simulink model "r2_b16a4x64f"  (R2012b)
settings: Solver=VariableStepDiscrete  SolverMode=SingleTasking  StartTime=0.0  StopTime=1  RelTol=1e-3
undefined symbols (not defined in the file): fft_stages, n_bits_ants, n_bits_xengs
libraries: xbsIndex_r4 x26846, casper_library_misc x230, xbsReplacements_r4 x24, casper_library_delays x8, xps_library x5, casper_library_communications x4
(part 37 of 227)

== system r2_b16a4x64f/sys0/xeng ==
  sync_in : Inport
  ant : Inport  Port=2
  window_valid : Inport  Port=3
  mcnt_in : Inport  Port=4
  Constant : xbsIndex_r4/Constant  const=0  gui_display_data_type=Fixed-point  arith_type=Unsigned  n_bits=200  bin_pt=14  preci_type=Single  exp_width=8  frac_width=24  explicit_period=on  period=1  equ=P=C  opselect=C  inp2=PCIN>>17  opr=+  inp1=P  carry=CIN  dbl_ovrd=off  block_type=constant
  Constant1 : xbsIndex_r4/Constant  const=0  gui_display_data_type=Fixed-point  arith_type=Boolean  n_bits=1  bin_pt=14  preci_type=Single  exp_width=8  frac_width=24  explicit_period=on  period=1  equ=P=C  opselect=C  inp2=PCIN>>17  opr=+  inp1=P  carry=CIN  dbl_ovrd=off  block_type=constant
  Term1 : Terminator
  Term2 : Terminator
  Term3 : Terminator
  auto_tap : Subsystem  AncestorBlock=casper_library_correlator/auto_tap  mask(auto_tap){n_ants=16, n_simultan=2, n_bits=8, acc_len=256, add_latency=3, mult_latency=4, bram_latency=7, mult_type=1, use_bram_delay=1}
      mask prompts: n_ants "Number of antennas (total inputs = n_ants*n_simultan below)"; n_simultan "Number of inputs fed-in simultaneously"; n_bits "Number of input bits (per complex component)"; acc_len "Accumulation length"; add_latency "Adder latency"; mult_latency "Multiplier latency"; bram_latency "BRAM latency"; mult_type "Multiplier Type (0=behavioural HDL, 1=embedded, 2=core)"; use_bram_delay "Implementation: Delay type (0=SLR, 1=BRAM)"
      mask init:
      | fix_pnt_pos = (n_bits-1)*2;
      | bit_growth = ceil(log2(acc_len));
      | ant_bits = ceil(log2(n_ants));
      | n_bits_out = (2*n_bits + 1 + bit_growth);
      | 
      | params = get_mask_params(gcb);
      | auto_tap_init(gcb, params{:});
      settings: AttributesFormatString=mult_typ=1, del_typ=1
  baseline_tap1 : Subsystem  AncestorBlock=casper_library_correlator/baseline_tap  mask(baseline_tap){n_ants=16, ant_sep=1, n_bits=8, acc_len=256, add_latency=3, mult_latency=4, bram_latency=7, mult_type=1, use_bram_delay=1}
      mask prompts: n_ants "Number of antennas"; ant_sep "Antenna Seperation"; n_bits "number of input bits (per complex component)"; acc_len "accumulation length"; add_latency "Adder latency"; mult_latency "Multiplier latency"; bram_latency "BRAM latency"; mult_type "Multiplier Type (0=behavioural HDL, 1=embedded, 2=core)"; use_bram_delay "Use BRAM delays"
      mask init:
      | fix_pnt_pos = (n_bits-1)*2;
      | bit_growth = ceil(log2(acc_len));
      | ant_bits = ceil(log2(n_ants));
      | n_bits_out = (2*n_bits + 1 + bit_growth);
      | 
      | params = get_mask_params(gcb);
      | baseline_tap_init(gcb, params{:});
      settings: AttributesFormatString=ant_sep=1, mult=1, bram=1
  baseline_tap2 : Subsystem  AncestorBlock=casper_library_correlator/baseline_tap  mask(baseline_tap){n_ants=16, ant_sep=2, n_bits=8, acc_len=256, add_latency=3, mult_latency=4, bram_latency=7, mult_type=1, use_bram_delay=1}
      mask prompts: n_ants "Number of antennas"; ant_sep "Antenna Seperation"; n_bits "number of input bits (per complex component)"; acc_len "accumulation length"; add_latency "Adder latency"; mult_latency "Multiplier latency"; bram_latency "BRAM latency"; mult_type "Multiplier Type (0=behavioural HDL, 1=embedded, 2=core)"; use_bram_delay "Use BRAM delays"
      mask init: same as r2_b16a4x64f/sys0/xeng/baseline_tap1
      settings: AttributesFormatString=ant_sep=2, mult=1, bram=1
  baseline_tap3 : Subsystem  AncestorBlock=casper_library_correlator/baseline_tap  mask(baseline_tap){n_ants=16, ant_sep=3, n_bits=8, acc_len=256, add_latency=3, mult_latency=4, bram_latency=7, mult_type=1, use_bram_delay=1}
      mask prompts: n_ants "Number of antennas"; ant_sep "Antenna Seperation"; n_bits "number of input bits (per complex component)"; acc_len "accumulation length"; add_latency "Adder latency"; mult_latency "Multiplier latency"; bram_latency "BRAM latency"; mult_type "Multiplier Type (0=behavioural HDL, 1=embedded, 2=core)"; use_bram_delay "Use BRAM delays"
      mask init: same as r2_b16a4x64f/sys0/xeng/baseline_tap1
      settings: AttributesFormatString=ant_sep=3, mult=1, bram=1
  baseline_tap4 : Subsystem  AncestorBlock=casper_library_correlator/baseline_tap  mask(baseline_tap){n_ants=16, ant_sep=4, n_bits=8, acc_len=256, add_latency=3, mult_latency=4, bram_latency=7, mult_type=1, use_bram_delay=1}
      mask prompts: n_ants "Number of antennas"; ant_sep "Antenna Seperation"; n_bits "number of input bits (per complex component)"; acc_len "accumulation length"; add_latency "Adder latency"; mult_latency "Multiplier latency"; bram_latency "BRAM latency"; mult_type "Multiplier Type (0=behavioural HDL, 1=embedded, 2=core)"; use_bram_delay "Use BRAM delays"
      mask init: same as r2_b16a4x64f/sys0/xeng/baseline_tap1
      settings: AttributesFormatString=ant_sep=4, mult=1, bram=1
  baseline_tap5 : Subsystem  AncestorBlock=casper_library_correlator/baseline_tap  mask(baseline_tap){n_ants=16, ant_sep=5, n_bits=8, acc_len=256, add_latency=3, mult_latency=4, bram_latency=7, mult_type=1, use_bram_delay=1}
      mask prompts: n_ants "Number of antennas"; ant_sep "Antenna Seperation"; n_bits "number of input bits (per complex component)"; acc_len "accumulation length"; add_latency "Adder latency"; mult_latency "Multiplier latency"; bram_latency "BRAM latency"; mult_type "Multiplier Type (0=behavioural HDL, 1=embedded, 2=core)"; use_bram_delay "Use BRAM delays"
      mask init: same as r2_b16a4x64f/sys0/xeng/baseline_tap1
      settings: AttributesFormatString=ant_sep=5, mult=1, bram=1
  baseline_tap6 : Subsystem  AncestorBlock=casper_library_correlator/baseline_tap  mask(baseline_tap){n_ants=16, ant_sep=6, n_bits=8, acc_len=256, add_latency=3, mult_latency=4, bram_latency=7, mult_type=1, use_bram_delay=1}
      mask prompts: n_ants "Number of antennas"; ant_sep "Antenna Seperation"; n_bits "number of input bits (per complex component)"; acc_len "accumulation length"; add_latency "Adder latency"; mult_latency "Multiplier latency"; bram_latency "BRAM latency"; mult_type "Multiplier Type (0=behavioural HDL, 1=embedded, 2=core)"; use_bram_delay "Use BRAM delays"
      mask init: same as r2_b16a4x64f/sys0/xeng/baseline_tap1
      settings: AttributesFormatString=ant_sep=6, mult=1, bram=1
  baseline_tap7 : Subsystem  AncestorBlock=casper_library_correlator/baseline_tap  mask(baseline_tap){n_ants=16, ant_sep=7, n_bits=8, acc_len=256, add_latency=3, mult_latency=4, bram_latency=7, mult_type=1, use_bram_delay=1}
      mask prompts: n_ants "Number of antennas"; ant_sep "Antenna Seperation"; n_bits "number of input bits (per complex component)"; acc_len "accumulation length"; add_latency "Adder latency"; mult_latency "Multiplier latency"; bram_latency "BRAM latency"; mult_type "Multiplier Type (0=behavioural HDL, 1=embedded, 2=core)"; use_bram_delay "Use BRAM delays"
      mask init: same as r2_b16a4x64f/sys0/xeng/baseline_tap1
      settings: AttributesFormatString=ant_sep=7, mult=1, bram=1
  baseline_tap8 : Subsystem  AncestorBlock=casper_library_correlator/baseline_tap  mask(baseline_tap){n_ants=16, ant_sep=8, n_bits=8, acc_len=256, add_latency=3, mult_latency=4, bram_latency=7, mult_type=1, use_bram_delay=1}
      mask prompts: n_ants "Number of antennas"; ant_sep "Antenna Seperation"; n_bits "number of input bits (per complex component)"; acc_len "accumulation length"; add_latency "Adder latency"; mult_latency "Multiplier latency"; bram_latency "BRAM latency"; mult_type "Multiplier Type (0=behavioural HDL, 1=embedded, 2=core)"; use_bram_delay "Use BRAM delays"
      mask init: same as r2_b16a4x64f/sys0/xeng/baseline_tap1
      settings: AttributesFormatString=ant_sep=8, mult=1, bram=1
  delay : xbsIndex_r4/Delay  rst=off  infoeditControl=Selection of Reset will increase slice count due to use of real FFs and instead of SRLs  en=off  latency=1  dbl_ovrd=off  reg_retiming=on  block_type=delay
  delay{1..3,5..6} (5 alike) : xbsIndex_r4/Delay  rst=off  infoeditControl=Selection of Reset will increase slice count due to use of real FFs and instead of SRLs  en=off  latency=3  dbl_ovrd=off  reg_retiming=on  block_type=delay
  sample_and_hold1 : Subsystem  AncestorBlock=casper_library_misc/sample_and_hold  mask(sample_and_hold){period=4096}
      mask prompts: period "Sample period (clocks)"
      mask help: This block will sample an input signal at a user specified rate and hold the value on the output.
  sample_and_hold2 : Subsystem  AncestorBlock=casper_library_misc/sample_and_hold  mask(sample_and_hold){period=4096}
      mask prompts: period "Sample period (clocks)"
      mask help: This block will sample an input signal at a user specified rate and hold the value on the output.
  sample_and_hold3 : Subsystem  AncestorBlock=casper_library_misc/sample_and_hold  mask(sample_and_hold){period=4096}
      mask prompts: period "Sample period (clocks)"
      mask help: This block will sample an input signal at a user specified rate and hold the value on the output.
  window_delay : casper_library_delays/window_delay  delay=273
  xeng_descramble : Subsystem  AncestorBlock=casper_library_correlator/xeng_descramble  mask(xeng_descramble){num_ants=16, n_bits=8, acc_len=256, demux_factor=4}
      mask prompts: num_ants "Number of Antennas"; n_bits "Input Bitwidth"; acc_len "X engine accumulation length"; demux_factor "Demux Factor"
      mask help:
      | NOT TESTED FOR non-2^N antennas.
      |
      | Descrambles X engine output. Optionally demuxes output.
      mask init:
      | num_taps = floor(num_ants/2) + 1;
      | ant_bits = ceil(log2(num_ants));
      | num_validins = num_ants*num_taps;
      | validin_bits = floor(log2(num_validins))+1;
      | demux_bits = floor(log2(demux_factor))+1;
      | acc_len_bits = floor(log2(acc_len))+1;
      | num_ants_bits = floor(log2(num_ants))+1;
      | taps_bits = floor(log2(num_taps))+1;
      | pivot_pnt = num_ants/2*(num_taps) + num_taps*num_ants/4;
      | num_elements = nchoosek(num_ants, 2) + num_ants;
      | elements_bits = floor(log2(num_elements)) + 1;
      | n_bits_xeng_out = (2*n_bits + acc_len_bits);
      | n_bits_in = 2^(ceil(log2(n_bits_xeng_out)))*8;
      | 
      | ship_el_del = floor(acc_len*num_ants/num_validins/demux_factor) - 1;
      | 
      | if (ship_el_del < 0)
      |     errordlg('Insufficient output space for this configuration. Try a lower demux setting. Else you need fewer antennas or longer xeng acc time.');
      |     ship_el_del=0;
      | end
      | 
      | if (ship_el_del == 0)
      |     ship_el_cnt = demux_factor*num_elements-1;
      |     %in this case we're outputting multiple words back-to-back.
      | else
      |     ship_el_cnt = demux_factor*num_elements;
      |     %in this case we're outputting one word at a time.
      | end
      | 
      | ship_el_del_bits = ceil(log2(ship_el_del + 1));
      | 
      | if (ship_el_del_bits == 0)
      |     ship_el_del_bits =1;
      | end
      | 
      | fmtstr = sprintf('num_ants=%d',num_ants);
      | set_param(gcb, 'AttributesFormatString', fmtstr);
      settings: AttributesFormatString=num_ants=16
  sync_out : Outport
  valid : Outport  Port=2
  acc : Outport  Port=3
  mcnt_out : Outport  Port=4
  wires:
  xeng_descramble/1(acc_out) -> acc/1
  xeng_descramble/2(valid_out) -> valid/1
  xeng_descramble/3(sync_out) -> sample_and_hold3/1(sync), sync_out/1
  baseline_tap8/4(acc_out) -> delay3/1
  baseline_tap8/5(valid_out) -> delay1/1
  baseline_tap8/7(sync_out) -> delay2/1
  window_delay/1 -> delay5/1
  ant/1 -> auto_tap/1(a_del), auto_tap/2(a_ndel)
  Constant/1 -> auto_tap/4(acc_in)
  Constant1/1 -> auto_tap/5(valid_in)
  sync_in/1 -> auto_tap/6(sync_in), sample_and_hold1/1(sync)
  window_valid/1 -> window_delay/1
  mcnt_in/1 -> sample_and_hold1/2(in)
  sample_and_hold1/1(out) -> delay6/1
  sample_and_hold2/1(out) -> sample_and_hold3/2(in)
  sample_and_hold3/1(out) -> delay/1
  delay/1 -> mcnt_out/1
  auto_tap/1(a_del_out) -> baseline_tap1/1(a_del)
  auto_tap/2(a_ndel_out) -> baseline_tap1/2(a_ndel)
  auto_tap/3(a_end_out) -> baseline_tap1/3(a_end)
  auto_tap/4(acc_out) -> baseline_tap1/4(acc_in)
  auto_tap/5(valid_out) -> baseline_tap1/5(valid_in)
  auto_tap/6(rst_out) -> baseline_tap1/6(rst)
  auto_tap/7(sync_out) -> baseline_tap1/7(sync1)
  baseline_tap1/1(a_del_out) -> baseline_tap2/1(a_del)
  baseline_tap1/2(a_ndel_out) -> baseline_tap2/2(a_ndel)
  baseline_tap1/3(a_end_out) -> baseline_tap2/3(a_end)
  baseline_tap1/4(acc_out) -> baseline_tap2/4(acc_in)
  baseline_tap1/5(valid_out) -> baseline_tap2/5(valid_in)
  baseline_tap1/6(rst_out) -> baseline_tap2/6(rst)
  baseline_tap1/7(sync_out) -> baseline_tap2/7(sync1)
  baseline_tap2/1(a_del_out) -> baseline_tap3/1(a_del)
  baseline_tap2/2(a_ndel_out) -> baseline_tap3/2(a_ndel)
  baseline_tap2/3(a_end_out) -> baseline_tap3/3(a_end)
  baseline_tap2/4(acc_out) -> baseline_tap3/4(acc_in)
  baseline_tap2/5(valid_out) -> baseline_tap3/5(valid_in)
  baseline_tap2/6(rst_out) -> baseline_tap3/6(rst)
  baseline_tap2/7(sync_out) -> baseline_tap3/7(sync1)
  baseline_tap3/1(a_del_out) -> baseline_tap4/1(a_del)
  baseline_tap3/2(a_ndel_out) -> baseline_tap4/2(a_ndel)
  baseline_tap3/3(a_end_out) -> baseline_tap4/3(a_end)
  baseline_tap3/4(acc_out) -> baseline_tap4/4(acc_in)
  baseline_tap3/5(valid_out) -> baseline_tap4/5(valid_in)
  baseline_tap3/6(rst_out) -> baseline_tap4/6(rst)
  baseline_tap3/7(sync_out) -> baseline_tap4/7(sync1)
  baseline_tap4/1(a_del_out) -> baseline_tap5/1(a_del)
  baseline_tap4/2(a_ndel_out) -> baseline_tap5/2(a_ndel)
  baseline_tap4/3(a_end_out) -> baseline_tap5/3(a_end)
  baseline_tap4/4(acc_out) -> baseline_tap5/4(acc_in)
  baseline_tap4/5(valid_out) -> baseline_tap5/5(valid_in)
  baseline_tap4/6(rst_out) -> baseline_tap5/6(rst)
  baseline_tap4/7(sync_out) -> baseline_tap5/7(sync1)
  baseline_tap5/1(a_del_out) -> baseline_tap6/1(a_del)
  baseline_tap5/2(a_ndel_out) -> baseline_tap6/2(a_ndel)
  baseline_tap5/3(a_end_out) -> baseline_tap6/3(a_end)
  baseline_tap5/4(acc_out) -> baseline_tap6/4(acc_in)
  baseline_tap5/5(valid_out) -> baseline_tap6/5(valid_in)
  baseline_tap5/6(rst_out) -> baseline_tap6/6(rst)
  baseline_tap5/7(sync_out) -> baseline_tap6/7(sync1)
  baseline_tap6/1(a_del_out) -> baseline_tap7/1(a_del)
  baseline_tap6/2(a_ndel_out) -> baseline_tap7/2(a_ndel)
  baseline_tap6/3(a_end_out) -> baseline_tap7/3(a_end)
  baseline_tap6/4(acc_out) -> baseline_tap7/4(acc_in)
  baseline_tap6/5(valid_out) -> baseline_tap7/5(valid_in)
  baseline_tap6/6(rst_out) -> baseline_tap7/6(rst)
  baseline_tap6/7(sync_out) -> baseline_tap7/7(sync1)
  baseline_tap7/1(a_del_out) -> baseline_tap8/1(a_del)
  baseline_tap7/2(a_ndel_out) -> baseline_tap8/2(a_ndel)
  baseline_tap7/3(a_end_out) -> baseline_tap8/3(a_end)
  baseline_tap7/4(acc_out) -> baseline_tap8/4(acc_in)
  baseline_tap7/5(valid_out) -> baseline_tap8/5(valid_in)
  baseline_tap7/6(rst_out) -> baseline_tap8/6(rst)
  baseline_tap7/7(sync_out) -> baseline_tap8/7(sync1)
  baseline_tap8/1(a_del_out) -> auto_tap/3(a_loop)
  baseline_tap8/2(a_ndel_out) -> Term1/1
  baseline_tap8/3(a_end_out) -> Term2/1
  baseline_tap8/6(rst_out) -> Term3/1
  delay1/1 -> xeng_descramble/2(valid)
  delay2/1 -> sample_and_hold2/1(sync), xeng_descramble/3(sync)
  delay3/1 -> xeng_descramble/1(acc)
  delay5/1 -> xeng_descramble/4(win_valid)
  delay6/1 -> sample_and_hold2/2(in)

== system r2_b16a4x64f/sys0/xeng_tvg ==
  tvg_sel : Inport
  sync : Inport  Port=2
  data_in : Inport  Port=3
  valid_in : Inport  Port=4
  mcnti : Inport  Port=5
  misci : Inport  Port=6
  Concat1 : xbsIndex_r4/Concat  num_inputs=4  dbl_ovrd=off  block_type=concat
      settings: block_version=10.1.3
  Constant1 : xbsIndex_r4/Constant  const=0.75  gui_display_data_type=Fixed-point  arith_type=Signed (2's comp)  n_bits=n_bits  bin_pt=n_bits-1  preci_type=Single  exp_width=8  frac_width=24  explicit_period=on  period=1  equ=P=C  opselect=C  inp2=PCIN>>17  opr=+  inp1=P  carry=CIN  dbl_ovrd=off  block_type=constant
  Constant13 : xbsIndex_r4/Constant  const=1  gui_display_data_type=Fixed-point  arith_type=Boolean  n_bits=1  bin_pt=0  preci_type=Single  exp_width=8  frac_width=24  explicit_period=on  period=1  equ=P=C  opselect=C  inp2=PCIN>>17  opr=+  inp1=P  carry=CIN  dbl_ovrd=off  block_type=constant
  Constant2 : xbsIndex_r4/Constant  const=0.125  gui_display_data_type=Fixed-point  arith_type=Signed (2's comp)  n_bits=n_bits  bin_pt=n_bits-1  preci_type=Single  exp_width=8  frac_width=24  explicit_period=on  period=1  equ=P=C  opselect=C  inp2=PCIN>>17  opr=+  inp1=P  carry=CIN  dbl_ovrd=off  block_type=constant
  Constant3 : xbsIndex_r4/Constant  const=0  gui_display_data_type=Fixed-point  arith_type=Unsigned  n_bits=2  bin_pt=0  preci_type=Single  exp_width=8  frac_width=24  explicit_period=on  period=1  equ=P=C  opselect=C  inp2=PCIN>>17  opr=+  inp1=P  carry=CIN  dbl_ovrd=off  block_type=constant
  Constant4 : xbsIndex_r4/Constant  const=-0.25  gui_display_data_type=Fixed-point  arith_type=Signed (2's comp)  n_bits=n_bits  bin_pt=n_bits-1  preci_type=Single  exp_width=8  frac_width=24  explicit_period=on  period=1  equ=P=C  opselect=C  inp2=PCIN>>17  opr=+  inp1=P  carry=CIN  dbl_ovrd=off  block_type=constant
  Constant7 : xbsIndex_r4/Constant  const=0.25  gui_display_data_type=Fixed-point  arith_type=Signed (2's comp)  n_bits=n_bits  bin_pt=n_bits-1  preci_type=Single  exp_width=8  frac_width=24  explicit_period=on  period=1  equ=P=C  opselect=C  inp2=PCIN>>17  opr=+  inp1=P  carry=CIN  dbl_ovrd=off  block_type=constant
  Counter : xbsIndex_r4/Counter  cnt_type=Free Running  cnt_to=Inf  operation=Up  start_count=0  cnt_by_val=1  arith_type=Unsigned  n_bits=x_int_bits + 1  bin_pt=0  load_pin=off  rst=on  en=off  explicit_period=off  period=1  dbl_ovrd=off  use_behavioral_HDL=off  implementation=Fabric  use_rpm=on  block_type=counter
      settings: xl_area=[0, 0, 0, 0, 0, 0, 0]
  Counter1 : xbsIndex_r4/Counter  cnt_type=Free Running  cnt_to=7  operation=Up  start_count=0  cnt_by_val=1  arith_type=Unsigned  n_bits=n_bits  bin_pt=0  load_pin=off  rst=on  en=on  explicit_period=off  period=1  dbl_ovrd=off  use_behavioral_HDL=off  implementation=Fabric  use_rpm=on  block_type=counter
      settings: xl_area=[0, 0, 0, 0, 0, 0, 0]
  Counter2 : xbsIndex_r4/Counter  cnt_type=Free Running  cnt_to=Inf  operation=Up  start_count=0  cnt_by_val=1  arith_type=Unsigned  n_bits=mcnt_period+1  bin_pt=0  load_pin=off  rst=on  en=on  explicit_period=off  period=1  dbl_ovrd=off  use_behavioral_HDL=off  implementation=Fabric  use_rpm=on  block_type=counter
      settings: xl_area=[0, 0, 0, 0, 0, 0, 0]
  Counter3 : xbsIndex_r4/Counter  cnt_type=Free Running  cnt_to=0  operation=Down  start_count=2^n_bits-1  cnt_by_val=1  arith_type=Unsigned  n_bits=n_bits  bin_pt=0  load_pin=off  rst=on  en=on  explicit_period=off  period=1  dbl_ovrd=off  use_behavioral_HDL=off  implementation=Fabric  use_rpm=on  block_type=counter
      settings: xl_area=[0, 0, 0, 0, 0, 0, 0]
  Counter4 : xbsIndex_r4/Counter  cnt_type=Free Running  cnt_to=Inf  operation=Up  start_count=2^sync_period - 2  cnt_by_val=1  arith_type=Unsigned  n_bits=sync_period+1  bin_pt=0  load_pin=off  rst=off  en=off  explicit_period=off  period=1  dbl_ovrd=off  use_behavioral_HDL=off  implementation=Fabric  use_rpm=on  block_type=counter
      settings: xl_area=[0, 0, 0, 0, 0, 0, 0]
  Counter5 : xbsIndex_r4/Counter  cnt_type=Free Running  cnt_to=Inf  operation=Up  start_count=0  cnt_by_val=mcnt_step  arith_type=Unsigned  n_bits=n_bits_mcnt  bin_pt=0  load_pin=off  rst=on  en=on  explicit_period=off  period=1  dbl_ovrd=off  use_behavioral_HDL=off  implementation=Fabric  use_rpm=on  block_type=counter
      settings: xl_area=[0, 0, 0, 0, 0, 0, 0]
  Delay{1,3..16} (15 alike) : xbsIndex_r4/Delay  rst=off  infoeditControl=Selection of Reset will increase slice count due to use of real FFs and instead of SRLs  en=off  latency=1  dbl_ovrd=off  reg_retiming=on  block_type=delay
      settings: xl_area=[0, 0, 0, 0, 0, 0, 0]
  Delay2 : xbsIndex_r4/Delay  rst=off  infoeditControl=Selection of Reset will increase slice count due to use of real FFs and instead of SRLs  en=off  latency=2  dbl_ovrd=off  reg_retiming=on  block_type=delay
      settings: xl_area=[0, 0, 0, 0, 0, 0, 0]
  Mux1 : xbsIndex_r4/Mux  inputs=2  en=off  latency=0  precision=Full  arith_type="Signed  (2's comp)"  n_bits=8  bin_pt=2  quantization=Truncate  overflow=Wrap  dbl_ovrd=off  block_type=mux
      settings: xl_area=[0, 0, 0, 0, 0, 0, 0]
  Mux2 : xbsIndex_r4/Mux  inputs=2  en=off  latency=1  precision=Full  arith_type="Signed  (2's comp)"  n_bits=8  bin_pt=2  quantization=Truncate  overflow=Wrap  dbl_ovrd=off  block_type=mux
      settings: xl_area=[0, 0, 0, 0, 0, 0, 0]
  Mux3 : xbsIndex_r4/Mux  inputs=4  en=off  latency=1  precision=Full  arith_type="Signed  (2's comp)"  n_bits=8  bin_pt=2  quantization=Truncate  overflow=Wrap  dbl_ovrd=off  block_type=mux
      settings: xl_area=[0, 0, 0, 0, 0, 0, 0]
  Mux4 : xbsIndex_r4/Mux  inputs=2  en=off  latency=0  precision=Full  arith_type="Signed  (2's comp)"  n_bits=8  bin_pt=2  quantization=Truncate  overflow=Wrap  dbl_ovrd=off  block_type=mux
      settings: xl_area=[0, 0, 0, 0, 0, 0, 0]
  Relational : xbsIndex_r4/Relational  mode=a!=b  en=off  latency=1  dbl_ovrd=off  block_type=relational
      settings: xl_area=[0, 0, 0, 0, 0, 0, 0]  block_version=10.1.3
  Slice1 : xbsIndex_r4/Slice  nbits=1  boolean_output=on  mode=Upper Bit Location + Width  bit1=0  base1=MSB of Input  bit0=x_int_bits  base0=LSB of Input  dbl_ovrd=off  block_type=slice
      settings: block_version=10.1.3
  Slice2 : xbsIndex_r4/Slice  nbits=1  boolean_output=on  mode=Lower Bit Location + Width  bit1=0  base1=MSB of Input  bit0=x_int_bits  base0=LSB of Input  dbl_ovrd=off  block_type=slice
      settings: infoedit="Extracts a given range of bits from each input sample and presents it at the output.  The output type is ordinarily unsigned with binary point at zero, but can be Boolean when the slice is one bit wide.<P><P>Hardware notes: In hardware this block costs nothing."  block_version=10.1.3
  Slice4 : xbsIndex_r4/Slice  nbits=1  boolean_output=on  mode=Lower Bit Location + Width  bit1=0  base1=MSB of Input  bit0=sync_period  base0=LSB of Input  dbl_ovrd=off  block_type=slice
      settings: infoedit="Extracts a given range of bits from each input sample and presents it at the output.  The output type is ordinarily unsigned with binary point at zero, but can be Boolean when the slice is one bit wide.<P><P>Hardware notes: In hardware this block costs nothing."  block_version=10.1.3
  ant_edge : Subsystem  AncestorBlock=casper_library_misc/edge_detect  mask(edge_detect){edge=Both, polarity=Active High, x_in=[0 0.08 0.08 0.16 0.16 0.24 0.24 0.32 0.32 0.4], y_in=[-1 -1  1  1  1  1  1  1  1  1], x_out=[0.6 0.68 0.68 0.76 0.76 0.84 0.84 0.92 0.92 1], y_out=[-1 -1  1  1 -1 -1 -1 -1 -1 -1]}
      mask prompts: edge "Edge Type"; polarity "Output Polarity"; x_in "Input X Positions"; y_in "Input Y Positions"; x_out "Output X Positions"; y_out "Output Y Positions"
      mask help: Output is active for one-cycle after each edge of the specified type (i.e. rising, falling or both).
      mask init: same as r2_b16a4x64f/edge_detect
      settings: AttributesFormatString=|
      | both edges
      | active high
      mask Help: Output is active for one-cycle after each edge of the specified type (i.e. rising, falling, or both).  Latency is zero.
      mask TypeOptions edge: Rising | Falling | Both
      mask TypeOptions polarity: Active High | Active Low
      mask Display:
      | plot(x_in_num,0.5+y_in_num*0.2);
      | plot(x_out_num,0.5+y_out_num*0.2);
  block_edge : Subsystem  AncestorBlock=casper_library_misc/edge_detect  mask(edge_detect){edge=Both, polarity=Active High, x_in=[0 0.08 0.08 0.16 0.16 0.24 0.24 0.32 0.32 0.4], y_in=[-1 -1  1  1  1  1  1  1  1  1], x_out=[0.6 0.68 0.68 0.76 0.76 0.84 0.84 0.92 0.92 1], y_out=[-1 -1  1  1 -1 -1 -1 -1 -1 -1]}
      mask prompts: edge "Edge Type"; polarity "Output Polarity"; x_in "Input X Positions"; y_in "Input Y Positions"; x_out "Output X Positions"; y_out "Output Y Positions"
      mask help: Output is active for one-cycle after each edge of the specified type (i.e. rising, falling or both).
      mask init: same as r2_b16a4x64f/edge_detect
      settings: AttributesFormatString=|
      | both edges
      | active high
      mask Help: Output is active for one-cycle after each edge of the specified type (i.e. rising, falling, or both).  Latency is zero.
      mask TypeOptions edge: Rising | Falling | Both
      mask TypeOptions polarity: Active High | Active Low
      mask Display:
      | plot(x_in_num,0.5+y_in_num*0.2);
      | plot(x_out_num,0.5+y_out_num*0.2);
  bus_create : Subsystem  AncestorBlock=casper_library_flow_control/bus_create  mask(bus_create){inputNum=4}
      mask prompts: inputNum "Number of inputs:"
      mask init:
      | bus_create_init(gcb,...
      |     'inputNum', inputNum);
  edge1 : Subsystem  AncestorBlock=casper_library_misc/edge_detect  mask(edge_detect){edge=Both, polarity=Active High, x_in=[0 0.08 0.08 0.16 0.16 0.24 0.24 0.32 0.32 0.4], y_in=[-1 -1  1  1  1  1  1  1  1  1], x_out=[0.6 0.68 0.68 0.76 0.76 0.84 0.84 0.92 0.92 1], y_out=[-1 -1  1  1 -1 -1 -1 -1 -1 -1]}
      mask prompts: edge "Edge Type"; polarity "Output Polarity"; x_in "Input X Positions"; y_in "Input Y Positions"; x_out "Output X Positions"; y_out "Output Y Positions"
      mask help: Output is active for one-cycle after each edge of the specified type (i.e. rising, falling or both).
      mask init: same as r2_b16a4x64f/edge_detect
      settings: AttributesFormatString=|
      | both edges
      | active high
      mask Help: Output is active for one-cycle after each edge of the specified type (i.e. rising, falling, or both).  Latency is zero.
      mask TypeOptions edge: Rising | Falling | Both
      mask TypeOptions polarity: Active High | Active Low
      mask Display:
      | plot(x_in_num,0.5+y_in_num*0.2);
      | plot(x_out_num,0.5+y_out_num*0.2);
  tvg_edge : Subsystem  AncestorBlock=casper_library_misc/edge_detect  mask(edge_detect){edge=Rising, polarity=Active High, x_in=[0 0.08 0.08 0.16 0.16 0.24 0.24 0.32 0.32 0.4], y_in=[-1 -1  1  1  1  1  1  1  1  1], x_out=[0.6 0.68 0.68 0.76 0.76 0.84 0.84 0.92 0.92 1], y_out=[-1 -1  1  1 -1 -1 -1 -1 -1 -1]}
      mask prompts: edge "Edge Type"; polarity "Output Polarity"; x_in "Input X Positions"; y_in "Input Y Positions"; x_out "Output X Positions"; y_out "Output Y Positions"
      mask help: Output is active for one-cycle after each edge of the specified type (i.e. rising, falling or both).
      mask init: same as r2_b16a4x64f/edge_detect
      settings: AttributesFormatString=|
      | rising edges
      | active high
      mask Help: Output is active for one-cycle after each edge of the specified type (i.e. rising, falling, or both).  Latency is zero.
      mask TypeOptions edge: Rising | Falling | Both
      mask TypeOptions polarity: Active High | Active Low
      mask Display:
      | plot(x_in_num,0.5+y_in_num*0.2);
      | plot(x_out_num,0.5+y_out_num*0.2);
  sync_out : Outport
  data_out : Outport  Port=2
  valid_out : Outport  Port=3
  mcnto : Outport  Port=4
  misco : Outport  Port=5
  wires:
  Constant2/1 -> bus_create/4(in4)
  Constant1/1 -> bus_create/2(in2)
  Constant7/1 -> bus_create/1(in1)
  Constant4/1 -> bus_create/3(in3)
  Counter1/1 -> Concat1/1, Concat1/3
  Slice2/1 -> ant_edge/1(in)
  Counter/1 -> Slice2/1
  Concat1/1 -> Delay4/1
  Delay7/1 -> sync_out/1
  data_in/1 -> Delay2/1
  Delay2/1 -> Mux3/2
  Mux3/1 -> data_out/1
  tvg_sel/1 -> Delay6/1, Relational/1
  Delay6/1 -> Mux3/1
  Constant3/1 -> Relational/2
  bus_create/1(bus_out) -> Mux3/4, Mux3/5
  Counter3/1 -> Concat1/2, Concat1/4
  Delay1/1 -> Delay7/1
  Delay8/1 -> Counter1/1, Counter3/1, Delay1/1
  Delay4/1 -> Mux3/3
  Relational/1 -> Delay10/1
  [use_tvg] -> Mux4/1
  Slice4/1 -> edge1/1(in)
  Counter4/1 -> Slice4/1
  sync/1 -> Mux4/2
  Mux4/1 -> Delay8/1, Counter/1
  edge1/1(out) -> Mux4/3
  Delay5/1 -> valid_out/1
  valid_in/1 -> Mux1/2
  Mux1/1 -> Delay9/1
  [use_tvg] -> Mux1/1
  Delay9/1 -> Counter2/2, Delay3/1
  Delay10/1 -> [use_tvg]
  mcnti/1 -> Delay14/1
  Mux2/1 -> mcnto/1
  Constant13/1 -> Mux1/3
  Delay15/1 -> Mux2/2
  Delay3/1 -> Delay5/1
  Delay14/1 -> Delay15/1
  tvg_edge/1(out) -> Counter5/1, Counter2/1
  [use_tvg] -> Mux2/1
  ant_edge/1(out) -> Counter1/2, Counter3/2
  [use_tvg] -> tvg_edge/1(in)
  Counter2/1 -> Slice1/1
  Counter5/1 -> Mux2/3
  Slice1/1 -> Delay11/1
  block_edge/1(out) -> Counter5/2
  Delay11/1 -> block_edge/1(in)
  misci/1 -> Delay12/1
  Delay12/1 -> Delay13/1
  Delay13/1 -> Delay16/1
  Delay16/1 -> misco/1

== system r2_b16a4x64f/sys0/zeros ==
  bus_create : Subsystem  AncestorBlock=casper_library_flow_control/bus_create  mask(bus_create){inputNum=19}
      mask prompts: inputNum "Number of inputs:"
      mask init:
      | bus_create_init(gcb,...
      |     'inputNum', inputNum);
  constant{0..18} (19 alike) : xbsIndex_r4/Constant  const=0  gui_display_data_type=Fixed-point  arith_type=Unsigned  n_bits=1  bin_pt=0  preci_type=Single  exp_width=8  frac_width=24  explicit_period=on  period=1  equ=P=C  opselect=C  inp2=PCIN>>17  opr=+  inp1=P  carry=CIN  dbl_ovrd=off  block_type=constant
  dout : Outport
  wires:
  constant0/1 -> bus_create/1(in1)
  constant1/1 -> bus_create/2(in2)
  constant2/1 -> bus_create/3(in3)
  constant3/1 -> bus_create/4(in4)
  constant4/1 -> bus_create/5(in5)
  constant5/1 -> bus_create/6(in6)
  constant6/1 -> bus_create/7(in7)
  constant7/1 -> bus_create/8(in8)
  constant8/1 -> bus_create/9(in9)
  constant9/1 -> bus_create/10(in10)
  constant10/1 -> bus_create/11(in11)
  constant11/1 -> bus_create/12(in12)
  constant12/1 -> bus_create/13(in13)
  constant13/1 -> bus_create/14(in14)
  constant14/1 -> bus_create/15(in15)
  constant15/1 -> bus_create/16(in16)
  constant16/1 -> bus_create/17(in17)
  constant17/1 -> bus_create/18(in18)
  constant18/1 -> bus_create/19(in19)
  bus_create/1(bus_out) -> dout/1

== system r2_b16a4x64f/sys1/Delay10 ==
  d : Inport
  Register0 : xbsIndex_r4/Register  init=0  rst=off  en=off  dbl_ovrd=off  block_type=register
      settings: block_version=11.4
  Register1 : xbsIndex_r4/Register  init=0  rst=off  en=off  dbl_ovrd=off  block_type=register
  q : Outport
  wires:
  Register1/1 -> q/1
  d/1 -> Register0/1
  Register0/1 -> Register1/1

== system r2_b16a4x64f/sys1/Delay11 ==
  d : Inport
  Register0 : xbsIndex_r4/Register  init=0  rst=off  en=off  dbl_ovrd=off  block_type=register
      settings: block_version=11.4
  Register1 : xbsIndex_r4/Register  init=0  rst=off  en=off  dbl_ovrd=off  block_type=register
  q : Outport
  wires:
  Register0/1 -> Register1/1
  d/1 -> Register0/1
  Register1/1 -> q/1

== system r2_b16a4x64f/sys1/Delay111 ==
  d : Inport
  Register0 : xbsIndex_r4/Register  init=0  rst=off  en=off  dbl_ovrd=off  block_type=register
      settings: block_version=11.4
  Register1 : xbsIndex_r4/Register  init=0  rst=off  en=off  dbl_ovrd=off  block_type=register
  q : Outport
  wires:
  Register1/1 -> q/1
  d/1 -> Register0/1
  Register0/1 -> Register1/1

== system r2_b16a4x64f/sys1/Delay12 ==
  d : Inport
  Register0 : xbsIndex_r4/Register  init=0  rst=off  en=off  dbl_ovrd=off  block_type=register
      settings: block_version=11.4
  Register1 : xbsIndex_r4/Register  init=0  rst=off  en=off  dbl_ovrd=off  block_type=register
  q : Outport
  wires:
  Register1/1 -> q/1
  d/1 -> Register0/1
  Register0/1 -> Register1/1

== system r2_b16a4x64f/sys1/Delay13 ==
  d : Inport
  Register0 : xbsIndex_r4/Register  init=0  rst=off  en=off  dbl_ovrd=off  block_type=register
      settings: block_version=11.4
  Register1 : xbsIndex_r4/Register  init=0  rst=off  en=off  dbl_ovrd=off  block_type=register
  q : Outport
  wires:
  Register0/1 -> Register1/1
  d/1 -> Register0/1
  Register1/1 -> q/1

== system r2_b16a4x64f/sys1/Delay14 ==
  d : Inport
  Register0 : xbsIndex_r4/Register  init=0  rst=off  en=off  dbl_ovrd=off  block_type=register
      settings: block_version=11.4
  Register1 : xbsIndex_r4/Register  init=0  rst=off  en=off  dbl_ovrd=off  block_type=register
  q : Outport
  wires:
  Register1/1 -> q/1
  d/1 -> Register0/1
  Register0/1 -> Register1/1

== system r2_b16a4x64f/sys1/Delay15 ==
  d : Inport
  Register0 : xbsIndex_r4/Register  init=0  rst=off  en=off  dbl_ovrd=off  block_type=register
      settings: block_version=11.4
  Register1 : xbsIndex_r4/Register  init=0  rst=off  en=off  dbl_ovrd=off  block_type=register
  q : Outport
  wires:
  Register1/1 -> q/1
  d/1 -> Register0/1
  Register0/1 -> Register1/1

== system r2_b16a4x64f/sys1/Delay16 ==
  d : Inport
  Register0 : xbsIndex_r4/Register  init=0  rst=off  en=off  dbl_ovrd=off  block_type=register
      settings: block_version=11.4
  Register1 : xbsIndex_r4/Register  init=0  rst=off  en=off  dbl_ovrd=off  block_type=register
  q : Outport
  wires:
  Register0/1 -> Register1/1
  d/1 -> Register0/1
  Register1/1 -> q/1

== system r2_b16a4x64f/sys1/Delay17 ==
  d : Inport
  Register0 : xbsIndex_r4/Register  init=0  rst=off  en=off  dbl_ovrd=off  block_type=register
      settings: block_version=11.4
  Register1 : xbsIndex_r4/Register  init=0  rst=off  en=off  dbl_ovrd=off  block_type=register
  q : Outport
  wires:
  Register1/1 -> q/1
  d/1 -> Register0/1
  Register0/1 -> Register1/1

== system r2_b16a4x64f/sys1/Delay18 ==
  d : Inport
  Register0 : xbsIndex_r4/Register  init=0  rst=off  en=off  dbl_ovrd=off  block_type=register
      settings: block_version=11.4
  Register1 : xbsIndex_r4/Register  init=0  rst=off  en=off  dbl_ovrd=off  block_type=register
  q : Outport
  wires:
  Register1/1 -> q/1
  d/1 -> Register0/1
  Register0/1 -> Register1/1

== system r2_b16a4x64f/sys1/Delay19 ==
  d : Inport
  Register0 : xbsIndex_r4/Register  init=0  rst=off  en=off  dbl_ovrd=off  block_type=register
      settings: block_version=11.4
  Register1 : xbsIndex_r4/Register  init=0  rst=off  en=off  dbl_ovrd=off  block_type=register
  q : Outport
  wires:
  Register0/1 -> Register1/1
  d/1 -> Register0/1
  Register1/1 -> q/1

== system r2_b16a4x64f/sys1/Delay20 ==
  d : Inport
  Register0 : xbsIndex_r4/Register  init=0  rst=off  en=off  dbl_ovrd=off  block_type=register
      settings: block_version=11.4
  Register1 : xbsIndex_r4/Register  init=0  rst=off  en=off  dbl_ovrd=off  block_type=register
  q : Outport
  wires:
  Register0/1 -> Register1/1
  d/1 -> Register0/1
  Register1/1 -> q/1

== system r2_b16a4x64f/sys1/Delay21 ==
  d : Inport
  Register0 : xbsIndex_r4/Register  init=0  rst=off  en=off  dbl_ovrd=off  block_type=register
      settings: block_version=11.4
  Register1 : xbsIndex_r4/Register  init=0  rst=off  en=off  dbl_ovrd=off  block_type=register
  q : Outport
  wires:
  Register1/1 -> q/1
  d/1 -> Register0/1
  Register0/1 -> Register1/1

== system r2_b16a4x64f/sys1/Delay22 ==
  d : Inport
  Register0 : xbsIndex_r4/Register  init=0  rst=off  en=off  dbl_ovrd=off  block_type=register
      settings: block_version=11.4
  Register1 : xbsIndex_r4/Register  init=0  rst=off  en=off  dbl_ovrd=off  block_type=register
  q : Outport
  wires:
  Register0/1 -> Register1/1
  d/1 -> Register0/1
  Register1/1 -> q/1

== system r2_b16a4x64f/sys1/Delay23 ==
  d : Inport
  Register0 : xbsIndex_r4/Register  init=0  rst=off  en=off  dbl_ovrd=off  block_type=register
      settings: block_version=11.4
  Register1 : xbsIndex_r4/Register  init=0  rst=off  en=off  dbl_ovrd=off  block_type=register
  q : Outport
  wires:
  Register1/1 -> q/1
  d/1 -> Register0/1
  Register0/1 -> Register1/1

== system r2_b16a4x64f/sys1/Delay24 ==
  d : Inport
  Register0 : xbsIndex_r4/Register  init=0  rst=off  en=off  dbl_ovrd=off  block_type=register
      settings: block_version=11.4
  Register1 : xbsIndex_r4/Register  init=0  rst=off  en=off  dbl_ovrd=off  block_type=register
  q : Outport
  wires:
  Register0/1 -> Register1/1
  d/1 -> Register0/1
  Register1/1 -> q/1

== system r2_b16a4x64f/sys1/Delay25 ==
  d : Inport
  Register0 : xbsIndex_r4/Register  init=0  rst=off  en=off  dbl_ovrd=off  block_type=register
      settings: block_version=11.4
  Register1 : xbsIndex_r4/Register  init=0  rst=off  en=off  dbl_ovrd=off  block_type=register
  q : Outport
  wires:
  Register1/1 -> q/1
  d/1 -> Register0/1
  Register0/1 -> Register1/1

== system r2_b16a4x64f/sys1/Delay26 ==
  d : Inport
  Register0 : xbsIndex_r4/Register  init=0  rst=off  en=off  dbl_ovrd=off  block_type=register
      settings: block_version=11.4
  Register1 : xbsIndex_r4/Register  init=0  rst=off  en=off  dbl_ovrd=off  block_type=register
  q : Outport
  wires:
  Register0/1 -> Register1/1
  d/1 -> Register0/1
  Register1/1 -> q/1

== system r2_b16a4x64f/sys1/Delay27 ==
  d : Inport
  Register0 : xbsIndex_r4/Register  init=0  rst=off  en=off  dbl_ovrd=off  block_type=register
      settings: block_version=11.4
  Register1 : xbsIndex_r4/Register  init=0  rst=off  en=off  dbl_ovrd=off  block_type=register
  q : Outport
  wires:
  Register0/1 -> Register1/1
  d/1 -> Register0/1
  Register1/1 -> q/1

== system r2_b16a4x64f/sys1/Delay28 ==
  d : Inport
  Register0 : xbsIndex_r4/Register  init=0  rst=off  en=off  dbl_ovrd=off  block_type=register
      settings: block_version=11.4
  Register1 : xbsIndex_r4/Register  init=0  rst=off  en=off  dbl_ovrd=off  block_type=register
  q : Outport
  wires:
  Register1/1 -> q/1
  d/1 -> Register0/1
  Register0/1 -> Register1/1

== system r2_b16a4x64f/sys1/Delay29 ==
  d : Inport
  Register0 : xbsIndex_r4/Register  init=0  rst=off  en=off  dbl_ovrd=off  block_type=register
      settings: block_version=11.4
  Register1 : xbsIndex_r4/Register  init=0  rst=off  en=off  dbl_ovrd=off  block_type=register
  q : Outport
  wires:
  Register1/1 -> q/1
  d/1 -> Register0/1
  Register0/1 -> Register1/1

== system r2_b16a4x64f/sys1/Delay35 ==
  d : Inport
  Register0 : xbsIndex_r4/Register  init=0  rst=off  en=off  dbl_ovrd=off  block_type=register
      settings: block_version=11.4
  q : Outport
  wires:
  Register0/1 -> q/1
  d/1 -> Register0/1

== system r2_b16a4x64f/sys1/Delay36 ==
  d : Inport
  Register0 : xbsIndex_r4/Register  init=0  rst=off  en=off  dbl_ovrd=off  block_type=register
      settings: block_version=11.4
  Register1 : xbsIndex_r4/Register  init=0  rst=off  en=off  dbl_ovrd=off  block_type=register
  q : Outport
  wires:
  Register0/1 -> Register1/1
  d/1 -> Register0/1
  Register1/1 -> q/1

== system r2_b16a4x64f/sys1/Delay37 ==
  d : Inport
  Register0 : xbsIndex_r4/Register  init=0  rst=off  en=off  dbl_ovrd=off  block_type=register
      settings: block_version=11.4
  q : Outport
  wires:
  Register0/1 -> q/1
  d/1 -> Register0/1

== system r2_b16a4x64f/sys1/Delay38 ==
  d : Inport
  Register0 : xbsIndex_r4/Register  init=0  rst=off  en=off  dbl_ovrd=off  block_type=register
      settings: block_version=11.4
  q : Outport
  wires:
  d/1 -> Register0/1
  Register0/1 -> q/1

== system r2_b16a4x64f/sys1/Delay39 ==
  d : Inport
  Register0 : xbsIndex_r4/Register  init=0  rst=off  en=off  dbl_ovrd=off  block_type=register
      settings: block_version=11.4
  q : Outport
  wires:
  Register0/1 -> q/1
  d/1 -> Register0/1

== system r2_b16a4x64f/sys1/Delay40 ==
  d : Inport
  Register0 : xbsIndex_r4/Register  init=0  rst=off  en=off  dbl_ovrd=off  block_type=register
      settings: block_version=11.4
  Register1 : xbsIndex_r4/Register  init=0  rst=off  en=off  dbl_ovrd=off  block_type=register
  q : Outport
  wires:
  Register1/1 -> q/1
  d/1 -> Register0/1
  Register0/1 -> Register1/1

== system r2_b16a4x64f/sys1/Delay41 ==
  d : Inport
  Register0 : xbsIndex_r4/Register  init=0  rst=off  en=off  dbl_ovrd=off  block_type=register
      settings: block_version=11.4
  Register1 : xbsIndex_r4/Register  init=0  rst=off  en=off  dbl_ovrd=off  block_type=register
  q : Outport
  wires:
  Register0/1 -> Register1/1
  d/1 -> Register0/1
  Register1/1 -> q/1

== system r2_b16a4x64f/sys1/Delay42 ==
  d : Inport
  Register0 : xbsIndex_r4/Register  init=0  rst=off  en=off  dbl_ovrd=off  block_type=register
      settings: block_version=11.4
  Register1 : xbsIndex_r4/Register  init=0  rst=off  en=off  dbl_ovrd=off  block_type=register
  q : Outport
  wires:
  Register0/1 -> Register1/1
  d/1 -> Register0/1
  Register1/1 -> q/1

== system r2_b16a4x64f/sys1/Delay43 ==
  d : Inport
  Register0 : xbsIndex_r4/Register  init=0  rst=off  en=off  dbl_ovrd=off  block_type=register
      settings: block_version=11.4
  Register1 : xbsIndex_r4/Register  init=0  rst=off  en=off  dbl_ovrd=off  block_type=register
  q : Outport
  wires:
  Register1/1 -> q/1
  d/1 -> Register0/1
  Register0/1 -> Register1/1

== system r2_b16a4x64f/sys1/Delay44 ==
  d : Inport
  Register0 : xbsIndex_r4/Register  init=0  rst=off  en=off  dbl_ovrd=off  block_type=register
      settings: block_version=11.4
  Register1 : xbsIndex_r4/Register  init=0  rst=off  en=off  dbl_ovrd=off  block_type=register
  q : Outport
  wires:
  Register0/1 -> Register1/1
  d/1 -> Register0/1
  Register1/1 -> q/1

== system r2_b16a4x64f/sys1/Delay45 ==
  d : Inport
  Register0 : xbsIndex_r4/Register  init=0  rst=off  en=off  dbl_ovrd=off  block_type=register
      settings: block_version=11.4
  Register1 : xbsIndex_r4/Register  init=0  rst=off  en=off  dbl_ovrd=off  block_type=register
  q : Outport
  wires:
  Register1/1 -> q/1
  d/1 -> Register0/1
  Register0/1 -> Register1/1

== system r2_b16a4x64f/sys1/Delay46 ==
  d : Inport
  Register0 : xbsIndex_r4/Register  init=0  rst=off  en=off  dbl_ovrd=off  block_type=register
      settings: block_version=11.4
  Register1 : xbsIndex_r4/Register  init=0  rst=off  en=off  dbl_ovrd=off  block_type=register
  q : Outport
  wires:
  Register0/1 -> Register1/1
  d/1 -> Register0/1
  Register1/1 -> q/1

== system r2_b16a4x64f/sys1/Delay47 ==
  d : Inport
  Register0 : xbsIndex_r4/Register  init=0  rst=off  en=off  dbl_ovrd=off  block_type=register
      settings: block_version=11.4
  Register1 : xbsIndex_r4/Register  init=0  rst=off  en=off  dbl_ovrd=off  block_type=register
  q : Outport
  wires:
  Register0/1 -> Register1/1
  d/1 -> Register0/1
  Register1/1 -> q/1

== system r2_b16a4x64f/sys1/Delay48 ==
  d : Inport
  Register0 : xbsIndex_r4/Register  init=0  rst=off  en=off  dbl_ovrd=off  block_type=register
      settings: block_version=11.4
  Register1 : xbsIndex_r4/Register  init=0  rst=off  en=off  dbl_ovrd=off  block_type=register
  q : Outport
  wires:
  Register0/1 -> Register1/1
  d/1 -> Register0/1
  Register1/1 -> q/1

== system r2_b16a4x64f/sys1/Delay49 ==
  d : Inport
  Register0 : xbsIndex_r4/Register  init=0  rst=off  en=off  dbl_ovrd=off  block_type=register
      settings: block_version=11.4
  Register1 : xbsIndex_r4/Register  init=0  rst=off  en=off  dbl_ovrd=off  block_type=register
  q : Outport
  wires:
  Register0/1 -> Register1/1
  d/1 -> Register0/1
  Register1/1 -> q/1

== system r2_b16a4x64f/sys1/Delay50 ==
  d : Inport
  Register0 : xbsIndex_r4/Register  init=0  rst=off  en=off  dbl_ovrd=off  block_type=register
      settings: block_version=11.4
  Register1 : xbsIndex_r4/Register  init=0  rst=off  en=off  dbl_ovrd=off  block_type=register
  q : Outport
  wires:
  Register1/1 -> q/1
  d/1 -> Register0/1
  Register0/1 -> Register1/1

== system r2_b16a4x64f/sys1/Delay51 ==
  d : Inport
  Register0 : xbsIndex_r4/Register  init=0  rst=off  en=off  dbl_ovrd=off  block_type=register
      settings: block_version=11.4
  Register1 : xbsIndex_r4/Register  init=0  rst=off  en=off  dbl_ovrd=off  block_type=register
  q : Outport
  wires:
  Register1/1 -> q/1
  d/1 -> Register0/1
  Register0/1 -> Register1/1

== system r2_b16a4x64f/sys1/Delay52 ==
  d : Inport
  Register0 : xbsIndex_r4/Register  init=0  rst=off  en=off  dbl_ovrd=off  block_type=register
      settings: block_version=11.4
  q : Outport
  wires:
  d/1 -> Register0/1
  Register0/1 -> q/1

== system r2_b16a4x64f/sys1/Delay53 ==
  d : Inport
  Register0 : xbsIndex_r4/Register  init=0  rst=off  en=off  dbl_ovrd=off  block_type=register
      settings: block_version=11.4
  Register1 : xbsIndex_r4/Register  init=0  rst=off  en=off  dbl_ovrd=off  block_type=register
  q : Outport
  wires:
  Register0/1 -> Register1/1
  d/1 -> Register0/1
  Register1/1 -> q/1

== system r2_b16a4x64f/sys1/Delay54 ==
  d : Inport
  Register0 : xbsIndex_r4/Register  init=0  rst=off  en=off  dbl_ovrd=off  block_type=register
      settings: block_version=11.4
  Register1 : xbsIndex_r4/Register  init=0  rst=off  en=off  dbl_ovrd=off  block_type=register
  q : Outport
  wires:
  Register1/1 -> q/1
  d/1 -> Register0/1
  Register0/1 -> Register1/1

== system r2_b16a4x64f/sys1/Delay55 ==
  d : Inport
  Register0 : xbsIndex_r4/Register  init=0  rst=off  en=off  dbl_ovrd=off  block_type=register
      settings: block_version=11.4
  Register1 : xbsIndex_r4/Register  init=0  rst=off  en=off  dbl_ovrd=off  block_type=register
  q : Outport
  wires:
  Register0/1 -> Register1/1
  d/1 -> Register0/1
  Register1/1 -> q/1

== system r2_b16a4x64f/sys1/Delay56 ==
  d : Inport
  Register0 : xbsIndex_r4/Register  init=0  rst=off  en=off  dbl_ovrd=off  block_type=register
      settings: block_version=11.4
  Register1 : xbsIndex_r4/Register  init=0  rst=off  en=off  dbl_ovrd=off  block_type=register
  q : Outport
  wires:
  Register1/1 -> q/1
  d/1 -> Register0/1
  Register0/1 -> Register1/1

== system r2_b16a4x64f/sys1/Delay57 ==
  d : Inport
  Register0 : xbsIndex_r4/Register  init=0  rst=off  en=off  dbl_ovrd=off  block_type=register
      settings: block_version=11.4
  Register1 : xbsIndex_r4/Register  init=0  rst=off  en=off  dbl_ovrd=off  block_type=register
  q : Outport
  wires:
  Register0/1 -> Register1/1
  d/1 -> Register0/1
  Register1/1 -> q/1

== system r2_b16a4x64f/sys1/Delay58 ==
  d : Inport
  Register0 : xbsIndex_r4/Register  init=0  rst=off  en=off  dbl_ovrd=off  block_type=register
      settings: block_version=11.4
  Register1 : xbsIndex_r4/Register  init=0  rst=off  en=off  dbl_ovrd=off  block_type=register
  q : Outport
  wires:
  Register1/1 -> q/1
  d/1 -> Register0/1
  Register0/1 -> Register1/1

== system r2_b16a4x64f/sys1/Delay59 ==
  d : Inport
  Register0 : xbsIndex_r4/Register  init=0  rst=off  en=off  dbl_ovrd=off  block_type=register
      settings: block_version=11.4
  Register1 : xbsIndex_r4/Register  init=0  rst=off  en=off  dbl_ovrd=off  block_type=register
  q : Outport
  wires:
  Register0/1 -> Register1/1
  d/1 -> Register0/1
  Register1/1 -> q/1

== system r2_b16a4x64f/sys1/Delay60 ==
  d : Inport
  Register0 : xbsIndex_r4/Register  init=0  rst=off  en=off  dbl_ovrd=off  block_type=register
      settings: block_version=11.4
  Register1 : xbsIndex_r4/Register  init=0  rst=off  en=off  dbl_ovrd=off  block_type=register
  q : Outport
  wires:
  Register1/1 -> q/1
  d/1 -> Register0/1
  Register0/1 -> Register1/1

== system r2_b16a4x64f/sys1/Delay61 ==
  d : Inport
  Register0 : xbsIndex_r4/Register  init=0  rst=off  en=off  dbl_ovrd=off  block_type=register
      settings: block_version=11.4
  Register1 : xbsIndex_r4/Register  init=0  rst=off  en=off  dbl_ovrd=off  block_type=register
  q : Outport
  wires:
  Register0/1 -> Register1/1
  d/1 -> Register0/1
  Register1/1 -> q/1

== system r2_b16a4x64f/sys1/Delay62 ==
  d : Inport
  Register0 : xbsIndex_r4/Register  init=0  rst=off  en=off  dbl_ovrd=off  block_type=register
      settings: block_version=11.4
  Register1 : xbsIndex_r4/Register  init=0  rst=off  en=off  dbl_ovrd=off  block_type=register
  q : Outport
  wires:
  Register1/1 -> q/1
  d/1 -> Register0/1
  Register0/1 -> Register1/1

== system r2_b16a4x64f/sys1/Delay69 ==
  d : Inport
  Register0 : xbsIndex_r4/Register  init=0  rst=off  en=off  dbl_ovrd=off  block_type=register
      settings: block_version=11.4
  Register1 : xbsIndex_r4/Register  init=0  rst=off  en=off  dbl_ovrd=off  block_type=register
      settings: block_version=11.4
  q : Outport
  wires:
  Register1/1 -> q/1
  d/1 -> Register0/1
  Register0/1 -> Register1/1

== system r2_b16a4x64f/sys1/Delay74 ==
  d : Inport
  Register0 : xbsIndex_r4/Register  init=0  rst=off  en=off  dbl_ovrd=off  block_type=register
      settings: block_version=11.4
  Register1 : xbsIndex_r4/Register  init=0  rst=off  en=off  dbl_ovrd=off  block_type=register
      settings: block_version=11.4
  q : Outport
  wires:
  Register1/1 -> q/1
  d/1 -> Register0/1
  Register0/1 -> Register1/1

== system r2_b16a4x64f/sys1/Delay76 ==
  d : Inport
  Register0 : xbsIndex_r4/Register  init=0  rst=off  en=off  dbl_ovrd=off  block_type=register
      settings: block_version=11.4
  Register1 : xbsIndex_r4/Register  init=0  rst=off  en=off  dbl_ovrd=off  block_type=register
      settings: block_version=11.4
  q : Outport
  wires:
  Register1/1 -> q/1
  d/1 -> Register0/1
  Register0/1 -> Register1/1

== system r2_b16a4x64f/sys1/Delay77 ==
  d : Inport
  Register0 : xbsIndex_r4/Register  init=0  rst=off  en=off  dbl_ovrd=off  block_type=register
      settings: block_version=11.4
  Register1 : xbsIndex_r4/Register  init=0  rst=off  en=off  dbl_ovrd=off  block_type=register
      settings: block_version=11.4
  q : Outport
  wires:
  Register0/1 -> Register1/1
  d/1 -> Register0/1
  Register1/1 -> q/1
